simulink model "Motor_Speed_Control_Block_Unit_Test"  (R2023b)
settings: Solver=VariableStepAuto  StartTime=0.0  StopTime=inf  RelTol=1e-3
undefined symbols (not defined in the file): Shooter_Error_Integral_Enable
libraries: simulink x1, Controls_Components_lib x1
settings Model: Creator=FIRSTMentor  LastModifiedBy=FIRSTMentor

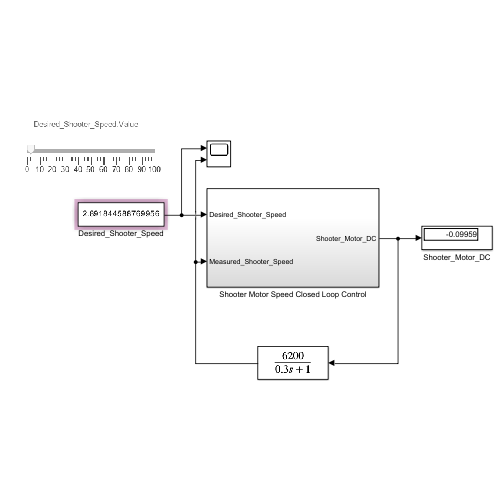
[thumbnail: Simulink's stored preview of the top-level diagram]
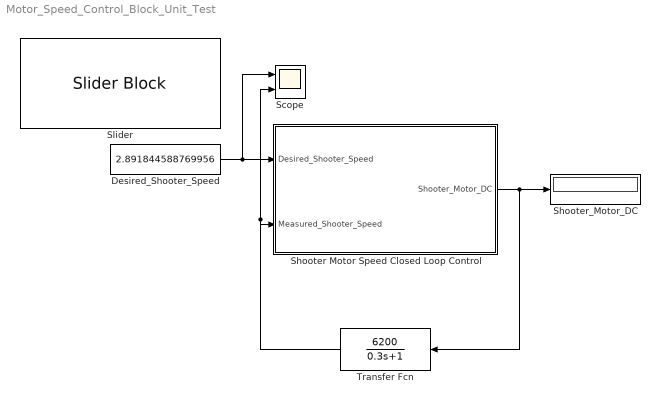
== system Motor_Speed_Control_Block_Unit_Test ==
  Desired_Shooter_Speed : Constant  Value=2.891844588769956
  Scope : Scope  NumInputPorts=2
  Shooter Motor Speed Closed Loop Control : Subsystem
  Shooter_Motor_DC : Display
  Slider : SliderBlock
  Transfer Fcn : TransferFcn  Numerator=[6200]  Denominator=[0.3 1]
  wires:
  Desired_Shooter_Speed/1 -> Scope/1, Shooter Motor Speed Closed Loop Control/1(Desired_Shooter_Speed)
  Shooter Motor Speed Closed Loop Control/1(Shooter_Motor_DC) -> Shooter_Motor_DC/1, Transfer Fcn/1
  Transfer Fcn/1 -> Scope/2, Shooter Motor Speed Closed Loop Control/2(Measured_Shooter_Speed)

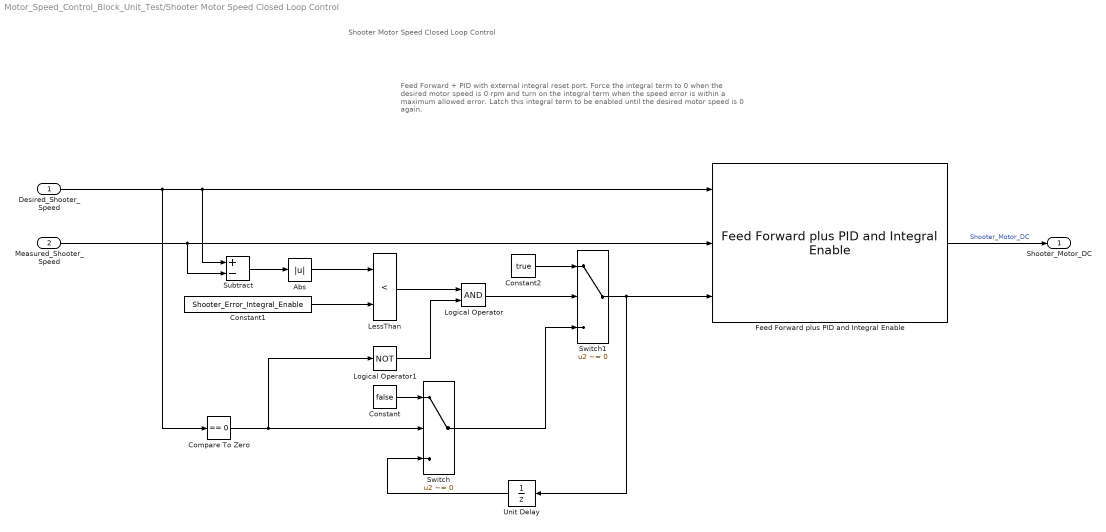
== system Motor_Speed_Control_Block_Unit_Test/Shooter Motor Speed Closed Loop Control ==
  note: Shooter Motor Speed Closed Loop Control
  note: Feed Forward + PID with external integral reset port.
      |
      | Force the integral term to 0 when the desired motor speed is 0 rpm and turn on the integral term when the speed error is within a maximum allowed error.  Latch this integral term to be enabled until the desired motor speed is 0 again.
  Desired_Shooter_Speed : Inport
  Measured_Shooter_Speed : Inport  Port=2
  Abs : Abs  SaturateOnIntegerOverflow=off
  Compare To Zero : simulink/Logic and Bit Operations/Compare To Zero  relop===  OutDataTypeStr=boolean
  Constant : Constant  Value=false
  Constant1 : Constant  Value=Shooter_Error_Integral_Enable
  Constant2 : Constant  Value=true
  Feed Forward plus PID and Integral Enable : Controls_Components_lib/Feed Forward plus PID and Integral Enable  Gain_FF=Shooter_Motor_Gain_FF  Gain_P=Shooter_Motor_Gain_P  Gain_I=Shooter_Motor_Gain_I  Gain_D=Shooter_Motor_Gain_D  FilterCoeff_D=0.1  Limit_I_Upper=0.1  Limit_I_Lower=-0.1  Limit_D_Upper=0.1  Limit_D_Lower=-0.1  Limit_T_Upper=1  Limit_T_Lower=-1
  LessThan : RelationalOperator  Operator=<  OutDataTypeStr=boolean  RndMeth=Simplest  InputSameDT=off
  Logical Operator : Logic  AllPortsSameDT=off  OutDataTypeStr=boolean
  Logical Operator1 : Logic  Operator=NOT  AllPortsSameDT=off  OutDataTypeStr=boolean
  Subtract : Sum  Inputs=+-
  Switch : Switch  Criteria=u2 ~= 0  SaturateOnIntegerOverflow=off  InputSameDT=off
  Switch1 : Switch  Criteria=u2 ~= 0  SaturateOnIntegerOverflow=off  InputSameDT=off
  Unit Delay : UnitDelay  SampleTime=-1  HasFrameUpgradeWarning=on
  Shooter_Motor_DC : Outport
  wires:
  Logical Operator1/1 -> Logical Operator/2
  Logical Operator/1 -> Switch1/2
  LessThan/1 -> Logical Operator/1
  Feed Forward plus PID and Integral Enable/1 -> Shooter_Motor_DC/1  "Shooter_Motor_DC"
  Subtract/1 -> Abs/1
  Constant1/1 -> LessThan/2
  Abs/1 -> LessThan/1
  Measured_Shooter_Speed/1 -> Subtract/2, Feed Forward plus PID and Integral Enable/2
  Desired_Shooter_Speed/1 -> Compare To Zero/1, Feed Forward plus PID and Integral Enable/1, Subtract/1
  Compare To Zero/1 -> Switch/2, Logical Operator1/1
  Constant/1 -> Switch/1
  Constant2/1 -> Switch1/1
  Switch1/1 -> Unit Delay/1, Feed Forward plus PID and Integral Enable/3
  Switch/1 -> Switch1/3
  Unit Delay/1 -> Switch/3
